simulink model "gtm_design"  (R2021b)
settings: Solver=ode15s  StartTime=0.0  StopTime=15  FixedStep=0.005  MaxStep=0.005  MinStep=0.0025
StopFcn:
  | MWSout=grabmws(bdroot);
  | MWSout.lastrun=datestr(now);
values from neighbouring files (symbols this model uses):
  s = tf('s')    [SingleDOF.m]    (also in main.m; newmain.m)
undefined symbols (not defined in the file or in its folder): Aero, aftfuel, aftfuel_pos, AILL, AILLC, AILR, AILRC, alpha_deg, altitude_ft, Ax_g, Ay_g, Az_g, b, beta_deg, bias, BRAKEC, Cbar, cg_pos0, cg_shift_gear, DamageCase, DamageModels, DamageOnsetTime, Earth, ELLIB, ELLIBC, ELLOB, ELLOBC, ELRIB, ELRIBC, ELROB, ELROBC, engl_ang, engl_pos, engr_ang, engr_pos, FLAPLIB, FLAPLIC, FLAPLOB, FLAPLOC, FLAPRIB, FLAPRIC, FLAPROB, FLAPROC, ft, FuelUsed_Init, fwdfuel, fwdfuel_pos, GEAR, GEARC, Inertia0, Inertia_shift_gear, Ixx_model, Iyy_model, Izz_model, KTAS, LandingGear, LengON, LinearizeModeOn, NAV_altitude_m, NAV_latitude_deg ... (+51)
libraries: simulink_extras x64, simulink_need_slupdate x30, LPVBlockLibrary x23, aerolibconvert2 x6, aerolibtransform2 x5, uavalgslib x4, UserContent_lib x3, simulink x3, robotcorelib x1, uavutilslib x1
(part 7 of 8)

== system gtm_design/GTM_T2/Sensors/Surface Pots/Sensor Model5 ==
  In1 : Inport
  Add : Sum  Inputs=+++
  Gain : Gain  Gain=scf
  Gear1 : Constant  Value=bias
  Gear2 : Constant  Value=noise_on
  Noise_on : Switch  Threshold=0.5  SaturateOnIntegerOverflow=on  InputSameDT=on
  White Noise : RandomNumber  Variance=sigma*sigma  Seed=round(seed*rand(1))  SampleTime=Timestep
  Out1 : Outport
  wires:
  Noise_on/1 -> Out1/1
  Gear2/1 -> Noise_on/2
  White Noise/1 -> Add/1
  Add/1 -> Noise_on/1
  Gear1/1 -> Add/2
  Gain/1 -> Add/3
  In1/1 -> Noise_on/3, Gain/1

== system gtm_design/GTM_T2/Sensors/Surface Pots/Surface Labels ==
  I : Inport
  Bus Creator : BusCreator  Inputs=12
  Demux : Demux  Outputs=12
  O : Outport
  wires:
  Bus Creator/1 -> O/1
  Demux/12 -> Bus Creator/12  "FLAPROB"
  Demux/11 -> Bus Creator/11  "FLAPRIB"
  Demux/10 -> Bus Creator/10  "FLAPLOB"
  Demux/9 -> Bus Creator/9  "FLAPLIB"
  Demux/8 -> Bus Creator/8  "RUDL"
  Demux/7 -> Bus Creator/7  "RUDU"
  Demux/6 -> Bus Creator/6  "AILR"
  Demux/5 -> Bus Creator/5  "AILL"
  Demux/4 -> Bus Creator/4  "ELRIB"
  Demux/3 -> Bus Creator/3  "ELROB"
  Demux/2 -> Bus Creator/2  "ELLIB"
  Demux/1 -> Bus Creator/1  "ELLOB"
  I/1 -> Demux/1

== system gtm_design/GTM_T2/TransportDelay/AntiAliasing/First Order Filter Continuous ==
  In : Inport
  Constant : Constant  Value=tau
  Divide : Product  Inputs=*/
  Integrator : Integrator  InitialConditionSource=external
  Sum : Sum  Inputs=-+|  InputSameDT=on  SaturateOnIntegerOverflow=on  OutDataTypeStr=Inherit: Same as first input
  Out : Outport
  wires:
  Constant/1 -> Divide/2
  Sum/1 -> Divide/1  "Error"
  In/1 -> Integrator/2, Sum/2
  Integrator/1 -> Out/1, Sum/1  "Y"
  Divide/1 -> Integrator/1  "Ydot"

== system gtm_design/GTM_T2/TransportDelay/Transport Delay on Bus/BusDelay ==
  In1 : Inport
  Bus Assignment : BusAssignment  AssignedSignals=alpha_deg,beta_deg,qbar_psf,KTAS,TEMPAMB_degF,altitude_ft
  Bus Selector1 : BusSelector  OutputSignals=alpha_deg,beta_deg,qbar_psf,KTAS,TEMPAMB_degF,altitude_ft  OutputAsBus=on
  Bus to Vector : BusToVector
  Demux : Demux  Outputs=6
  TimeDelay with IC feedthrough : Subsystem  mask{TimeDelay=15e-3}
      mask prompts: TimeDelay "Time Delay (sec)"
      mask help:
      | Implements Continuous Time Transport Delay with initial
      | outputs set to feedthrough with no delay.
      |
      |   output = input;   for t<TimeDelay
      |   output = input(t-tdelay); for t>=TimeDelay
  Out1 : Outport
  wires:
  In1/1 -> Bus Assignment/1, Bus Selector1/1
  Bus Selector1/1 -> Bus to Vector/1
  Bus to Vector/1 -> TimeDelay with IC feedthrough/1(I)
  TimeDelay with IC feedthrough/1(O) -> Demux/1
  Demux/1 -> Bus Assignment/2
  Demux/2 -> Bus Assignment/3
  Demux/3 -> Bus Assignment/4
  Demux/4 -> Bus Assignment/5
  Demux/5 -> Bus Assignment/6
  Demux/6 -> Bus Assignment/7
  Bus Assignment/1 -> Out1/1

== system gtm_design/GTM_T2/TransportDelay/Transport Delay on Bus/BusDelay1 ==
  In1 : Inport
  Bus Assignment : BusAssignment  AssignedSignals=phi_deg,theta_deg,psi_deg,NAV_latitude_deg,NAV_longitude_deg,NAV_altitude_m,NAV_Vn_mps,NAV_Ve_mps,NAV_Vu_mps
  Bus Selector1 : BusSelector  OutputSignals=phi_deg,theta_deg,psi_deg,NAV_latitude_deg,NAV_longitude_deg,NAV_altitude_m,NAV_Vn_mps,NAV_Ve_mps,NAV_Vu_mps  OutputAsBus=on
  Bus to Vector : BusToVector
  Demux : Demux  Outputs=9
  TimeDelay with IC feedthrough : Subsystem  mask{TimeDelay=15e-3}
      mask prompts: TimeDelay "Time Delay (sec)"
      mask help:
      | Implements Continuous Time Transport Delay with initial
      | outputs set to feedthrough with no delay.
      |
      |   output = input;   for t<TimeDelay
      |   output = input(t-tdelay); for t>=TimeDelay
  Out1 : Outport
  wires:
  In1/1 -> Bus Assignment/1, Bus Selector1/1
  Bus Selector1/1 -> Bus to Vector/1
  Bus to Vector/1 -> TimeDelay with IC feedthrough/1(I)
  TimeDelay with IC feedthrough/1(O) -> Demux/1
  Demux/1 -> Bus Assignment/2
  Demux/2 -> Bus Assignment/3
  Demux/3 -> Bus Assignment/4
  Demux/4 -> Bus Assignment/5
  Demux/5 -> Bus Assignment/6
  Demux/6 -> Bus Assignment/7
  Bus Assignment/1 -> Out1/1
  Demux/7 -> Bus Assignment/8
  Demux/8 -> Bus Assignment/9
  Demux/9 -> Bus Assignment/10

== system gtm_design/GTM_T2/TransportDelay/Transport Delay on Bus/BusDelay2 ==
  In1 : Inport
  Bus Assignment : BusAssignment  AssignedSignals=p_deg,q_deg,r_deg,Ax_g,Ay_g,Az_g
  Bus Selector1 : BusSelector  OutputSignals=p_deg,q_deg,r_deg,Ax_g,Ay_g,Az_g  OutputAsBus=on
  Bus to Vector : BusToVector
  Demux : Demux  Outputs=6
  TimeDelay with IC feedthrough : Subsystem  mask{TimeDelay=15e-3}
      mask prompts: TimeDelay "Time Delay (sec)"
      mask help:
      | Implements Continuous Time Transport Delay with initial
      | outputs set to feedthrough with no delay.
      |
      |   output = input;   for t<TimeDelay
      |   output = input(t-tdelay); for t>=TimeDelay
  Out1 : Outport
  wires:
  In1/1 -> Bus Assignment/1, Bus Selector1/1
  Bus Selector1/1 -> Bus to Vector/1
  Bus to Vector/1 -> TimeDelay with IC feedthrough/1(I)
  TimeDelay with IC feedthrough/1(O) -> Demux/1
  Demux/1 -> Bus Assignment/2
  Demux/2 -> Bus Assignment/3
  Demux/3 -> Bus Assignment/4
  Demux/4 -> Bus Assignment/5
  Demux/5 -> Bus Assignment/6
  Demux/6 -> Bus Assignment/7
  Bus Assignment/1 -> Out1/1

== system gtm_design/GTM_T2/TransportDelay/Transport Delay on Bus/BusDelay3 ==
  In1 : Inport
  Bus Assignment : BusAssignment  AssignedSignals=ELLOB,ELLIB,ELROB,ELRIB,AILL,AILR,RUDU,RUDL,FLAPLIB,FLAPLOB,FLAPRIB,FLAPROB
  Bus Selector1 : BusSelector  OutputSignals=ELLOB,ELLIB,ELROB,ELRIB,AILL,AILR,RUDU,RUDL,FLAPLIB,FLAPLOB,FLAPRIB,FLAPROB  OutputAsBus=on
  Bus to Vector : BusToVector
  Demux : Demux  Outputs=12
  TimeDelay with IC feedthrough : Subsystem  mask{TimeDelay=15e-3}
      mask prompts: TimeDelay "Time Delay (sec)"
      mask help:
      | Implements Continuous Time Transport Delay with initial
      | outputs set to feedthrough with no delay.
      |
      |   output = input;   for t<TimeDelay
      |   output = input(t-tdelay); for t>=TimeDelay
  Out1 : Outport
  wires:
  In1/1 -> Bus Assignment/1, Bus Selector1/1
  Bus Selector1/1 -> Bus to Vector/1
  Bus to Vector/1 -> TimeDelay with IC feedthrough/1(I)
  TimeDelay with IC feedthrough/1(O) -> Demux/1
  Bus Assignment/1 -> Out1/1
  Demux/1 -> Bus Assignment/2
  Demux/2 -> Bus Assignment/3
  Demux/3 -> Bus Assignment/4
  Demux/4 -> Bus Assignment/5
  Demux/5 -> Bus Assignment/6
  Demux/6 -> Bus Assignment/7
  Demux/7 -> Bus Assignment/8
  Demux/8 -> Bus Assignment/9
  Demux/9 -> Bus Assignment/10
  Demux/10 -> Bus Assignment/11
  Demux/11 -> Bus Assignment/12
  Demux/12 -> Bus Assignment/13

== system gtm_design/GTM_T2/TransportDelay/Transport Delay on Bus/BusDelay4 ==
  In1 : Inport
  Bus Assignment : BusAssignment  AssignedSignals=RPML,PUMPVL,RPMR,PUMPVR
  Bus Selector1 : BusSelector  OutputSignals=RPML,PUMPVL,RPMR,PUMPVR  OutputAsBus=on
  Bus to Vector : BusToVector
  Demux : Demux
  TimeDelay with IC feedthrough : Subsystem  mask{TimeDelay=15e-3}
      mask prompts: TimeDelay "Time Delay (sec)"
      mask help:
      | Implements Continuous Time Transport Delay with initial
      | outputs set to feedthrough with no delay.
      |
      |   output = input;   for t<TimeDelay
      |   output = input(t-tdelay); for t>=TimeDelay
  Out1 : Outport
  wires:
  In1/1 -> Bus Assignment/1, Bus Selector1/1
  Bus Selector1/1 -> Bus to Vector/1
  Bus to Vector/1 -> TimeDelay with IC feedthrough/1(I)
  TimeDelay with IC feedthrough/1(O) -> Demux/1
  Demux/1 -> Bus Assignment/2
  Demux/2 -> Bus Assignment/3
  Demux/3 -> Bus Assignment/4
  Demux/4 -> Bus Assignment/5
  Bus Assignment/1 -> Out1/1

== system gtm_design/GTM_T2/TransportDelay/Transport Delay on Bus1/BusDelay ==
  In1 : Inport
  Bus Assignment : BusAssignment  AssignedSignals=THROTLC,THROTRC,ELLOBC,ELLIBC,ELROBC,ELRIBC,AILLC,AILRC,RUDUPC,RUDLOC,SPLLIBC,SPLLOBC,SPLRIBC,SPLROBC,FLAPLIC,FLAPLOC,FLAPRIC,FLAPROC,GEARC,BRAKEC,STEERC
  Bus Selector1 : BusSelector  OutputSignals=THROTLC,THROTRC,ELLOBC,ELLIBC,ELROBC,ELRIBC,AILLC,AILRC,RUDUPC,RUDLOC,SPLLIBC,SPLLOBC,SPLRIBC,SPLROBC,FLAPLIC,FLAPLOC,FLAPRIC,FLAPROC,GEARC,BRAKEC,STEERC  OutputAsBus=on
  Bus to Vector : BusToVector
  Demux : Demux  Outputs=21
  Transport Delay : TransportDelay  DelayTime=5e-3
      settings: AttributesFormatString=%<DelayTime>
  Out1 : Outport
  wires:
  In1/1 -> Bus Assignment/1, Bus Selector1/1
  Bus Selector1/1 -> Bus to Vector/1
  Bus to Vector/1 -> Transport Delay/1
  Transport Delay/1 -> Demux/1
  Demux/1 -> Bus Assignment/2
  Demux/2 -> Bus Assignment/3
  Demux/3 -> Bus Assignment/4
  Demux/4 -> Bus Assignment/5
  Demux/5 -> Bus Assignment/6
  Demux/6 -> Bus Assignment/7
  Bus Assignment/1 -> Out1/1
  Demux/7 -> Bus Assignment/8
  Demux/8 -> Bus Assignment/9
  Demux/9 -> Bus Assignment/10
  Demux/10 -> Bus Assignment/11
  Demux/11 -> Bus Assignment/12
  Demux/12 -> Bus Assignment/13
  Demux/13 -> Bus Assignment/14
  Demux/14 -> Bus Assignment/15
  Demux/15 -> Bus Assignment/16
  Demux/16 -> Bus Assignment/17
  Demux/17 -> Bus Assignment/18
  Demux/18 -> Bus Assignment/19
  Demux/19 -> Bus Assignment/20
  Demux/20 -> Bus Assignment/21
  Demux/21 -> Bus Assignment/22

== system gtm_design/GTM_T2/A//C parameters/Inertia//Mass//CG Shift/FuelBurnEffects/Polyval ==
  In1 : Inport
  Embedded MATLAB Function : MATLAB Function  TreatAsAtomicUnit=on
  Out1 : Outport
  wires:
  In1/1 -> Embedded MATLAB Function/1(u)
  Embedded MATLAB Function/1(y) -> Out1/1

== system gtm_design/GTM_T2/A//C parameters/Inertia//Mass//CG Shift/FuelBurnEffects/Polyval1 ==
  In1 : Inport
  Embedded MATLAB Function : MATLAB Function  TreatAsAtomicUnit=on
  Out1 : Outport
  wires:
  In1/1 -> Embedded MATLAB Function/1(u)
  Embedded MATLAB Function/1(y) -> Out1/1

== system gtm_design/GTM_T2/A//C parameters/Inertia//Mass//CG Shift/FuelBurnEffects/Polyval2 ==
  In1 : Inport
  Embedded MATLAB Function : MATLAB Function  TreatAsAtomicUnit=on
  Out1 : Outport
  wires:
  In1/1 -> Embedded MATLAB Function/1(u)
  Embedded MATLAB Function/1(y) -> Out1/1

== system gtm_design/GTM_T2/Actuators/InputModification for Trimming/LinearizeMode:DetlasOnTrimBias/Surface Allocation For Linearizing ==
  I : Inport
  BiasSurfs : Subsystem
  Demux : Demux  Outputs=19
  Gain1 : Gain  Gain=-1
  Ground1 : Ground
  Ground2 : Ground
  Ground5 : Ground
  Mux : Mux  Inputs=22
  O : Outport
  wires:
  BiasSurfs/1(cmds) -> O/1
  I/1 -> Demux/1
  Mux/1 -> BiasSurfs/1(dCmd)
  Ground1/1 -> Mux/18  "dgear"
  Ground2/1 -> Mux/19  "dbrake"
  Ground5/1 -> Mux/22  "dSteer"
  Demux/1 -> Mux/1  "dElevatorLOB"
  Demux/2 -> Mux/2  "dElevatorLIB"
  Demux/3 -> Mux/3  "dElevatorROB"
  Demux/4 -> Mux/4  "dElevatorRIB"
  Demux/5 -> Gain1/1  "dAileronL"
  Demux/6 -> Mux/6  "dAileronR"
  Demux/7 -> Mux/7  "dRudderUpper"
  Demux/8 -> Mux/8  "dRudderLower"
  Demux/9 -> Mux/9  "dSpoilerLOB"
  Demux/10 -> Mux/10  "dSpoilerLIB"
  Demux/11 -> Mux/11  "dSpoilerRIB"
  Demux/12 -> Mux/12  "dSpoilerROB"
  Demux/13 -> Mux/13  "dFlapLIB"
  Demux/14 -> Mux/14  "dFlapLOB"
  Demux/15 -> Mux/15  "dFlapRIB"
  Demux/16 -> Mux/16  "dFlapROB"
  Demux/17 -> Mux/17  "dStabilizer"
  Demux/18 -> Mux/20  "dThrottleL"
  Demux/19 -> Mux/21  "dThrottleR"
  Gain1/1 -> Mux/5  "dAileronL"

== system gtm_design/GTM_T2/Actuators/InputModification for Trimming/TrimMode: DriveFromTopLevel/Force Consistent Sample Time on Bus ==
  In1 : Inport
  Bus to Vector : BusToVector
  Map4 : Gain
  Out1 : Outport
  wires:
  In1/1 -> Bus to Vector/1
  Map4/1 -> Out1/1
  Bus to Vector/1 -> Map4/1

== system gtm_design/GTM_T2/Actuators/InputModification for Trimming/TrimMode: DriveFromTopLevel/InitializeBus ==
  Bus Creator : BusCreator  Inputs=22
  Constant : Constant  Value=zeros(22,1)
  Demux : Demux  Outputs=22
  O : Outport
  wires:
  Constant/1 -> Demux/1
  Demux/18 -> Bus Creator/18  "GEAR"
  Demux/19 -> Bus Creator/19  "BRAKE"
  Demux/20 -> Bus Creator/20  "THROTL"
  Demux/21 -> Bus Creator/21  "THROTR"
  Demux/22 -> Bus Creator/22  "STEER"
  Demux/17 -> Bus Creator/17  "STAB"
  Bus Creator/1 -> O/1
  Demux/2 -> Bus Creator/2  "ELLIB"
  Demux/3 -> Bus Creator/3  "ELROB"
  Demux/4 -> Bus Creator/4  "ELRIB"
  Demux/5 -> Bus Creator/5  "AILL"
  Demux/6 -> Bus Creator/6  "AILR"
  Demux/7 -> Bus Creator/7  "RUDU"
  Demux/8 -> Bus Creator/8  "RUDL"
  Demux/9 -> Bus Creator/9  "SPLLIB"
  Demux/10 -> Bus Creator/10  "SPLLOB"
  Demux/11 -> Bus Creator/11  "SPLRIB"
  Demux/12 -> Bus Creator/12  "SPLROB"
  Demux/13 -> Bus Creator/13  "FLAPLIB"
  Demux/14 -> Bus Creator/14  "FLAPLOB"
  Demux/15 -> Bus Creator/15  "FLAPRIB"
  Demux/16 -> Bus Creator/16  "FLAPROB"
  Demux/1 -> Bus Creator/1  "ELLOB"

== system gtm_design/GTM_T2/Actuators/InputModification for Trimming/TrimMode: DriveFromTopLevel/MapPitchSurf ==
  UseStab : Inport
  In : Inport  Port=2
  Merge : Merge
  Switch Case : SwitchCase
  UseElevatorToTrim : Subsystem  TreatAsAtomicUnit=on
  UseStabToTrim : Subsystem  TreatAsAtomicUnit=on
  Out : Outport
  wires:
  UseElevatorToTrim/1(Out) -> Merge/1
  UseStabToTrim/1(Out1) -> Merge/2
  In/1 -> UseStabToTrim/1(In), UseElevatorToTrim/1(In)
  Merge/1 -> Out/1
  Switch Case/2 -> UseElevatorToTrim/Action
  UseStab/1 -> Switch Case/1
  Switch Case/1 -> UseStabToTrim/Action

== system gtm_design/GTM_T2/Aero/Basic Airframe/DamageEffects/Switch Case Action Subsystem ==
  alpha : Inport
  beta : Inport  Port=2
  damage_case : Inport  Port=3
  Action Port : ActionPort  ActionPortLabel=case [ 1 2 3 4 5 6 ]:
  AlphaLookup : PreLookup  BreakpointsData=Aero.dC6_damage.bas.alpha  BeginIndexSearchUsingPreviousIndexResult=on  ExtrapMethod=Linear
  BetaLookup : PreLookup  BreakpointsData=Aero.dC6_damage.bas.beta  ExtrapMethod=Linear
  Constant : Constant  Value=uint32(1)
  Constant4 : Constant  Value=[0:5]  OutDataTypeStr=uint32
  Interpolation Using Prelookup : Interpolation_n-D  NumberOfTableDimensions=4  Table=Aero.dC6_damage.bas.data  ExtrapMethod=Clip  NumSelectionDims=2
      settings: InputPortMap=u0,u1,u2,u3,u4,u5
  Subtract : Sum  Inputs=+-
  dC6_dam : Outport  InitialOutput=zeros(6,1)
  wires:
  Constant/1 -> Subtract/2
  Subtract/1 -> Interpolation Using Prelookup/5
  damage_case/1 -> Subtract/1
  BetaLookup/2 -> Interpolation Using Prelookup/4
  BetaLookup/1 -> Interpolation Using Prelookup/3
  AlphaLookup/2 -> Interpolation Using Prelookup/2
  AlphaLookup/1 -> Interpolation Using Prelookup/1
  Interpolation Using Prelookup/1 -> dC6_dam/1
  beta/1 -> BetaLookup/1
  alpha/1 -> AlphaLookup/1
  Constant4/1 -> Interpolation Using Prelookup/6

== system gtm_design/GTM_T2/Aero/Basic Airframe/DamageEffects/Switch Case Action Subsystem2 ==
  Action Port : ActionPort  ActionPortLabel=default:
  Constant4 : Constant  Value=zeros(6,1)  OutDataTypeStr=double
  Zeros : Outport  InitialOutput=zeros(6,1)
  wires:
  Constant4/1 -> Zeros/1

== system gtm_design/GTM_T2/Aero/Control Surfaces/Elevator//Stab1/RollYaw Coupling LIB ==
  I : Inport
  Gain : Gain  Gain=Kc  Multiplication=Matrix(K*u)
  O : Outport
  wires:
  Gain/1 -> O/1
  I/1 -> Gain/1

== system gtm_design/GTM_T2/Aero/Control Surfaces/Elevator//Stab1/RollYaw Coupling LOB ==
  I : Inport
  Gain : Gain  Gain=Kc  Multiplication=Matrix(K*u)
  O : Outport
  wires:
  Gain/1 -> O/1
  I/1 -> Gain/1

== system gtm_design/GTM_T2/Aero/Control Surfaces/Elevator//Stab1/RollYaw Coupling RIB ==
  I : Inport
  Gain : Gain  Gain=Kc  Multiplication=Matrix(K*u)
  O : Outport
  wires:
  Gain/1 -> O/1
  I/1 -> Gain/1

== system gtm_design/GTM_T2/Aero/Control Surfaces/Elevator//Stab1/RollYaw Coupling ROB ==
  I : Inport
  Gain : Gain  Gain=Kc  Multiplication=Matrix(K*u)
  O : Outport
  wires:
  Gain/1 -> O/1
  I/1 -> Gain/1

== system gtm_design/GTM_T2/Aero/Control Surfaces/Elevator//Stab1/Stab//Elev Table ==
  alpha_k : Inport
  alpha_f : Inport  Port=2
  beta_k : Inport  Port=3
  beta_f : Inport  Port=4
  stab_k : Inport  Port=5
  stab_f : Inport  Port=6
  elev : Inport  Port=7
  Assignment to Longitudinal : Assignment  IndexMode=Zero-based  IndexOptions=Index vector (dialog)  Indices=[0 2 4]  OutputSizes=[1 1]
  Constant : Constant  Value=zeros(6,1)
  Constant2 : Constant  Value=[0:2]  OutDataTypeStr=uint32
  Interpolation Using Prelookup : Interpolation_n-D  NumberOfTableDimensions=5  Table=Aero.dC3_ele.data  NumSelectionDims=1
      settings: InputPortMap=u0,u1,u2,u3,u4,u5,u6,u7,u8
  Prelookup4 : PreLookup  BreakpointsData=Aero.dC3_ele.elev  IndexSearchMethod=Linear search  BeginIndexSearchUsingPreviousIndexResult=on  ExtrapMethod=Linear
  dC6 : Outport
  wires:
  Constant2/1 -> Interpolation Using Prelookup/9
  Prelookup4/2 -> Interpolation Using Prelookup/8
  Prelookup4/1 -> Interpolation Using Prelookup/7
  stab_f/1 -> Interpolation Using Prelookup/6
  beta_f/1 -> Interpolation Using Prelookup/4
  alpha_f/1 -> Interpolation Using Prelookup/2
  alpha_k/1 -> Interpolation Using Prelookup/1
  beta_k/1 -> Interpolation Using Prelookup/3
  stab_k/1 -> Interpolation Using Prelookup/5
  elev/1 -> Prelookup4/1
  Constant/1 -> Assignment to Longitudinal/1
  Interpolation Using Prelookup/1 -> Assignment to Longitudinal/2
  Assignment to Longitudinal/1 -> dC6/1

== system gtm_design/GTM_T2/Aero/Control Surfaces/Elevator//Stab1/Stab//Elev Table0 ==
  alpha_k : Inport
  alpha_f : Inport  Port=2
  beta_k : Inport  Port=3
  beta_f : Inport  Port=4
  stab_k : Inport  Port=5
  stab_f : Inport  Port=6
  elev : Inport  Port=7
  Assignment to Longitudinal : Assignment  IndexMode=Zero-based  IndexOptions=Index vector (dialog)  Indices=[0 2 4]  OutputSizes=[1 1]
  Constant : Constant  Value=zeros(6,1)
  Constant2 : Constant  Value=[0:2]  OutDataTypeStr=uint32
  Interpolation Using Prelookup : Interpolation_n-D  NumberOfTableDimensions=5  Table=Aero.dC3_ele.data  NumSelectionDims=1
      settings: InputPortMap=u0,u1,u2,u3,u4,u5,u6,u7,u8
  Prelookup4 : PreLookup  BreakpointsData=Aero.dC3_ele.elev  IndexSearchMethod=Linear search  BeginIndexSearchUsingPreviousIndexResult=on  ExtrapMethod=Linear
  dC6 : Outport
  wires:
  Constant2/1 -> Interpolation Using Prelookup/9
  Prelookup4/2 -> Interpolation Using Prelookup/8
  Prelookup4/1 -> Interpolation Using Prelookup/7
  stab_f/1 -> Interpolation Using Prelookup/6
  beta_f/1 -> Interpolation Using Prelookup/4
  alpha_f/1 -> Interpolation Using Prelookup/2
  alpha_k/1 -> Interpolation Using Prelookup/1
  beta_k/1 -> Interpolation Using Prelookup/3
  stab_k/1 -> Interpolation Using Prelookup/5
  elev/1 -> Prelookup4/1
  Constant/1 -> Assignment to Longitudinal/1
  Interpolation Using Prelookup/1 -> Assignment to Longitudinal/2
  Assignment to Longitudinal/1 -> dC6/1

== system gtm_design/GTM_T2/Aero/Control Surfaces/Elevator//Stab1/Stab//Elev Table1 ==
  alpha_k : Inport
  alpha_f : Inport  Port=2
  beta_k : Inport  Port=3
  beta_f : Inport  Port=4
  stab_k : Inport  Port=5
  stab_f : Inport  Port=6
  elev : Inport  Port=7
  Assignment to Longitudinal : Assignment  IndexMode=Zero-based  IndexOptions=Index vector (dialog)  Indices=[0 2 4]  OutputSizes=[1 1]
  Constant : Constant  Value=zeros(6,1)
  Constant2 : Constant  Value=[0:2]  OutDataTypeStr=uint32
  Interpolation Using Prelookup : Interpolation_n-D  NumberOfTableDimensions=5  Table=Aero.dC3_ele.data  NumSelectionDims=1
      settings: InputPortMap=u0,u1,u2,u3,u4,u5,u6,u7,u8
  Prelookup4 : PreLookup  BreakpointsData=Aero.dC3_ele.elev  IndexSearchMethod=Linear search  BeginIndexSearchUsingPreviousIndexResult=on  ExtrapMethod=Linear
  dC6 : Outport
  wires:
  Constant2/1 -> Interpolation Using Prelookup/9
  Prelookup4/2 -> Interpolation Using Prelookup/8
  Prelookup4/1 -> Interpolation Using Prelookup/7
  stab_f/1 -> Interpolation Using Prelookup/6
  beta_f/1 -> Interpolation Using Prelookup/4
  alpha_f/1 -> Interpolation Using Prelookup/2
  alpha_k/1 -> Interpolation Using Prelookup/1
  beta_k/1 -> Interpolation Using Prelookup/3
  stab_k/1 -> Interpolation Using Prelookup/5
  elev/1 -> Prelookup4/1
  Constant/1 -> Assignment to Longitudinal/1
  Interpolation Using Prelookup/1 -> Assignment to Longitudinal/2
  Assignment to Longitudinal/1 -> dC6/1

== system gtm_design/GTM_T2/Aero/Control Surfaces/Elevator//Stab1/Stab//Elev Table2 ==
  alpha_k : Inport
  alpha_f : Inport  Port=2
  beta_k : Inport  Port=3
  beta_f : Inport  Port=4
  stab_k : Inport  Port=5
  stab_f : Inport  Port=6
  elev : Inport  Port=7
  Assignment to Longitudinal : Assignment  IndexMode=Zero-based  IndexOptions=Index vector (dialog)  Indices=[0 2 4]  OutputSizes=[1 1]
  Constant : Constant  Value=zeros(6,1)
  Constant2 : Constant  Value=[0:2]  OutDataTypeStr=uint32
  Interpolation Using Prelookup : Interpolation_n-D  NumberOfTableDimensions=5  Table=Aero.dC3_ele.data  NumSelectionDims=1
      settings: InputPortMap=u0,u1,u2,u3,u4,u5,u6,u7,u8
  Prelookup4 : PreLookup  BreakpointsData=Aero.dC3_ele.elev  IndexSearchMethod=Linear search  BeginIndexSearchUsingPreviousIndexResult=on  ExtrapMethod=Linear
  dC6 : Outport
  wires:
  Constant2/1 -> Interpolation Using Prelookup/9
  Prelookup4/2 -> Interpolation Using Prelookup/8
  Prelookup4/1 -> Interpolation Using Prelookup/7
  stab_f/1 -> Interpolation Using Prelookup/6
  beta_f/1 -> Interpolation Using Prelookup/4
  alpha_f/1 -> Interpolation Using Prelookup/2
  alpha_k/1 -> Interpolation Using Prelookup/1
  beta_k/1 -> Interpolation Using Prelookup/3
  stab_k/1 -> Interpolation Using Prelookup/5
  elev/1 -> Prelookup4/1
  Constant/1 -> Assignment to Longitudinal/1
  Interpolation Using Prelookup/1 -> Assignment to Longitudinal/2
  Assignment to Longitudinal/1 -> dC6/1

== system gtm_design/GTM_T2/Aero/Control Surfaces/Elevator//Stab1/Stab//Elev Table3 ==
  alpha_k : Inport
  alpha_f : Inport  Port=2
  beta_k : Inport  Port=3
  beta_f : Inport  Port=4
  stab_k : Inport  Port=5
  stab_f : Inport  Port=6
  elev : Inport  Port=7
  Assignment to Longitudinal : Assignment  IndexMode=Zero-based  IndexOptions=Index vector (dialog)  Indices=[0 2 4]  OutputSizes=[1 1]
  Constant : Constant  Value=zeros(6,1)
  Constant2 : Constant  Value=[0:2]  OutDataTypeStr=uint32
  Interpolation Using Prelookup : Interpolation_n-D  NumberOfTableDimensions=5  Table=Aero.dC3_ele.data  NumSelectionDims=1
      settings: InputPortMap=u0,u1,u2,u3,u4,u5,u6,u7,u8
  Prelookup4 : PreLookup  BreakpointsData=Aero.dC3_ele.elev  IndexSearchMethod=Linear search  BeginIndexSearchUsingPreviousIndexResult=on  ExtrapMethod=Linear
  dC6 : Outport
  wires:
  Constant2/1 -> Interpolation Using Prelookup/9
  Prelookup4/2 -> Interpolation Using Prelookup/8
  Prelookup4/1 -> Interpolation Using Prelookup/7
  stab_f/1 -> Interpolation Using Prelookup/6
  beta_f/1 -> Interpolation Using Prelookup/4
  alpha_f/1 -> Interpolation Using Prelookup/2
  alpha_k/1 -> Interpolation Using Prelookup/1
  beta_k/1 -> Interpolation Using Prelookup/3
  stab_k/1 -> Interpolation Using Prelookup/5
  elev/1 -> Prelookup4/1
  Constant/1 -> Assignment to Longitudinal/1
  Interpolation Using Prelookup/1 -> Assignment to Longitudinal/2
  Assignment to Longitudinal/1 -> dC6/1

== system gtm_design/GTM_T2/Aero/Control Surfaces/Rudder/Gains ==
  dC6_in : Inport
  Product : Product  RndMeth=Zero
  gains : Constant  Value=gains
  dC6 : Outport
  wires:
  dC6_in/1 -> Product/1
  Product/1 -> dC6/1
  gains/1 -> Product/2

== system gtm_design/GTM_T2/Aero/Control Surfaces/Rudder/Gains1 ==
  dC6_in : Inport
  Product : Product  RndMeth=Zero
  gains : Constant  Value=gains
  dC6 : Outport
  wires:
  gains/1 -> Product/2
  Product/1 -> dC6/1
  dC6_in/1 -> Product/1

== system gtm_design/GTM_T2/Aero/Control Surfaces/Rudder/Lower Rudder ==
  alpha : Inport
  beta : Inport  Port=2
  rud : Inport  Port=3
  Abs : Abs
  Assignment to lateral : Assignment  IndexMode=Zero-based  IndexOptions=Index vector (dialog)  Indices=[1 3 5]  OutputSizes=[1 1]
  Constant : Constant  Value=-1
  Constant1 : Constant
  Constant2 : Constant  Value=[0:5]  OutDataTypeStr=uint32
  Constant3 : Constant  Value=ones(6,1)
  Gain : Gain  Gain=-1
  Interpolation Using Prelookup : Interpolation_n-D  NumberOfTableDimensions=4  Table=Aero.dC6_rud.data  NumSelectionDims=1
      settings: InputPortMap=u0,u1,u2,u3,u4,u5,u6
  Prelookup : PreLookup  BreakpointsData=Aero.dC6_rud.alpha  IndexSearchMethod=Linear search  BeginIndexSearchUsingPreviousIndexResult=on  ExtrapMethod=Linear
  Prelookup1 : PreLookup  BreakpointsData=Aero.dC6_rud.beta  IndexSearchMethod=Linear search  BeginIndexSearchUsingPreviousIndexResult=on  ExtrapMethod=Linear
  Prelookup2 : PreLookup  BreakpointsData=Aero.dC6_rud.rud  IndexSearchMethod=Linear search  BeginIndexSearchUsingPreviousIndexResult=on  ExtrapMethod=Linear
  Product1 : Product  RndMeth=Zero
  Product2 : Product  RndMeth=Zero
  Switch : Switch
  dC6 : Outport
  wires:
  Interpolation Using Prelookup/1 -> Product2/1
  Assignment to lateral/1 -> Product2/2
  Constant3/1 -> Assignment to lateral/1
  Switch/1 -> Assignment to lateral/2, Product1/2
  Constant1/1 -> Switch/3
  Constant/1 -> Switch/1
  Product2/1 -> dC6/1
  beta/1 -> Product1/1
  alpha/1 -> Prelookup/1
  Gain/1 -> Prelookup2/1
  Abs/1 -> Gain/1
  rud/1 -> Switch/2, Abs/1
  Product1/1 -> Prelookup1/1
  Prelookup/1 -> Interpolation Using Prelookup/1
  Prelookup/2 -> Interpolation Using Prelookup/2
  Prelookup1/1 -> Interpolation Using Prelookup/3
  Prelookup1/2 -> Interpolation Using Prelookup/4
  Prelookup2/1 -> Interpolation Using Prelookup/5
  Prelookup2/2 -> Interpolation Using Prelookup/6
  Constant2/1 -> Interpolation Using Prelookup/7

== system gtm_design/GTM_T2/Aero/Control Surfaces/Rudder/Upper Rudder ==
  alpha : Inport
  beta : Inport  Port=2
  rud : Inport  Port=3
  Abs : Abs
  Assignment to lateral : Assignment  IndexMode=Zero-based  IndexOptions=Index vector (dialog)  Indices=[1 3 5]  OutputSizes=[1 1]
  Constant : Constant  Value=-1
  Constant1 : Constant
  Constant2 : Constant  Value=[0:5]  OutDataTypeStr=uint32
  Constant3 : Constant  Value=ones(6,1)
  Gain : Gain  Gain=-1
  Interpolation Using Prelookup : Interpolation_n-D  NumberOfTableDimensions=4  Table=Aero.dC6_rud.data  NumSelectionDims=1
      settings: InputPortMap=u0,u1,u2,u3,u4,u5,u6
  Prelookup : PreLookup  BreakpointsData=Aero.dC6_rud.alpha  IndexSearchMethod=Linear search  BeginIndexSearchUsingPreviousIndexResult=on  ExtrapMethod=Linear
  Prelookup1 : PreLookup  BreakpointsData=Aero.dC6_rud.beta  IndexSearchMethod=Linear search  BeginIndexSearchUsingPreviousIndexResult=on  ExtrapMethod=Linear
  Prelookup2 : PreLookup  BreakpointsData=Aero.dC6_rud.rud  IndexSearchMethod=Linear search  BeginIndexSearchUsingPreviousIndexResult=on  ExtrapMethod=Linear
  Product1 : Product  RndMeth=Zero
  Product2 : Product  RndMeth=Zero
  Switch : Switch
  dC6 : Outport
  wires:
  Constant2/1 -> Interpolation Using Prelookup/7
  Prelookup2/2 -> Interpolation Using Prelookup/6
  Prelookup2/1 -> Interpolation Using Prelookup/5
  Prelookup1/2 -> Interpolation Using Prelookup/4
  Prelookup1/1 -> Interpolation Using Prelookup/3
  Prelookup/2 -> Interpolation Using Prelookup/2
  Prelookup/1 -> Interpolation Using Prelookup/1
  Product1/1 -> Prelookup1/1
  rud/1 -> Abs/1, Switch/2
  Abs/1 -> Gain/1
  Gain/1 -> Prelookup2/1
  alpha/1 -> Prelookup/1
  beta/1 -> Product1/1
  Product2/1 -> dC6/1
  Constant/1 -> Switch/1
  Constant1/1 -> Switch/3
  Switch/1 -> Product1/2, Assignment to lateral/2
  Constant3/1 -> Assignment to lateral/1
  Assignment to lateral/1 -> Product2/2
  Interpolation Using Prelookup/1 -> Product2/1

== system gtm_design/GTM_T2/Aero/Control Surfaces/Spoilers/Gains1 ==
  dC6_in : Inport
  Product : Product  RndMeth=Zero
  gains : Constant  Value=gains
  dC6 : Outport
  wires:
  dC6_in/1 -> Product/1
  Product/1 -> dC6/1
  gains/1 -> Product/2

== system gtm_design/GTM_T2/Aero/Control Surfaces/Spoilers/Gains2 ==
  dC6_in : Inport
  Product : Product  RndMeth=Zero
  gains : Constant  Value=gains
  dC6 : Outport
  wires:
  gains/1 -> Product/2
  Product/1 -> dC6/1
  dC6_in/1 -> Product/1

== system gtm_design/GTM_T2/Aero/Control Surfaces/Spoilers/Gains3 ==
  dC6_in : Inport
  Product : Product  RndMeth=Zero
  gains : Constant  Value=gains
  dC6 : Outport
  wires:
  gains/1 -> Product/2
  Product/1 -> dC6/1
  dC6_in/1 -> Product/1

== system gtm_design/GTM_T2/Aero/Control Surfaces/Spoilers/Gains4 ==
  dC6_in : Inport
  Product : Product  RndMeth=Zero
  gains : Constant  Value=gains
  dC6 : Outport
  wires:
  dC6_in/1 -> Product/1
  Product/1 -> dC6/1
  gains/1 -> Product/2

== system gtm_design/GTM_T2/Aero/Control Surfaces/Spoilers/InboardSpoilers ==
  alpha : Inport
  beta : Inport  Port=2
  SPLLIB : Inport  Port=3
  SPLRIB : Inport  Port=4
  Constant1 : Constant  Value=[0:5]  OutDataTypeStr=uint32
  Constant3 : Constant  Value=[0:5]  OutDataTypeStr=uint32
  Gain2 : Gain  Gain=-1
  Interpolation Using Prelookup : Interpolation_n-D  NumberOfTableDimensions=4  Table=Aero.dC6_spo.data  NumSelectionDims=1
      settings: InputPortMap=u0,u1,u2,u3,u4,u5,u6
  Interpolation Using Prelookup1 : Interpolation_n-D  NumberOfTableDimensions=4  Table=Aero.dC6_spo.data  NumSelectionDims=1
      settings: InputPortMap=u0,u1,u2,u3,u4,u5,u6
  Negate Lateral : Gain  Gain=[1 -1 1 -1 1 -1]
  Prelookup1 : PreLookup  BreakpointsData=Aero.dC6_spo.alpha  IndexSearchMethod=Linear search  BeginIndexSearchUsingPreviousIndexResult=on  ExtrapMethod=Linear
  Prelookup2 : PreLookup  BreakpointsData=Aero.dC6_spo.beta  IndexSearchMethod=Linear search  BeginIndexSearchUsingPreviousIndexResult=on  ExtrapMethod=Linear
  Prelookup3 : PreLookup  BreakpointsData=Aero.dC6_spo.spo  IndexSearchMethod=Linear search  BeginIndexSearchUsingPreviousIndexResult=on  ExtrapMethod=Linear
  Prelookup4 : PreLookup  BreakpointsData=Aero.dC6_spo.beta  IndexSearchMethod=Linear search  BeginIndexSearchUsingPreviousIndexResult=on  ExtrapMethod=Linear
  Prelookup5 : PreLookup  BreakpointsData=Aero.dC6_spo.spo  IndexSearchMethod=Linear search  BeginIndexSearchUsingPreviousIndexResult=on  ExtrapMethod=Linear
  Left : Outport
  Right : Outport  Port=2
  wires:
  Gain2/1 -> Prelookup2/1
  Negate Lateral/1 -> Left/1
  Interpolation Using Prelookup1/1 -> Right/1
  SPLRIB/1 -> Prelookup5/1
  beta/1 -> Gain2/1, Prelookup4/1
  alpha/1 -> Prelookup1/1
  SPLLIB/1 -> Prelookup3/1
  Prelookup1/1 -> Interpolation Using Prelookup/1, Interpolation Using Prelookup1/1
  Prelookup1/2 -> Interpolation Using Prelookup/2, Interpolation Using Prelookup1/2
  Prelookup2/1 -> Interpolation Using Prelookup/3
  Prelookup2/2 -> Interpolation Using Prelookup/4
  Prelookup3/1 -> Interpolation Using Prelookup/5
  Prelookup3/2 -> Interpolation Using Prelookup/6
  Constant3/1 -> Interpolation Using Prelookup/7
  Prelookup4/1 -> Interpolation Using Prelookup1/3
  Prelookup4/2 -> Interpolation Using Prelookup1/4
  Prelookup5/1 -> Interpolation Using Prelookup1/5
  Prelookup5/2 -> Interpolation Using Prelookup1/6
  Constant1/1 -> Interpolation Using Prelookup1/7
  Interpolation Using Prelookup/1 -> Negate Lateral/1

== system gtm_design/GTM_T2/Aero/Control Surfaces/Spoilers/OutboardSpoilers ==
  alpha : Inport
  beta : Inport  Port=2
  SPLLIB : Inport  Port=3
  SPLRIB : Inport  Port=4
  Constant1 : Constant  Value=[0:5]  OutDataTypeStr=uint32
  Constant3 : Constant  Value=[0:5]  OutDataTypeStr=uint32
  Gain2 : Gain  Gain=-1
  Interpolation Using Prelookup : Interpolation_n-D  NumberOfTableDimensions=4  Table=Aero.dC6_spo.data  NumSelectionDims=1
      settings: InputPortMap=u0,u1,u2,u3,u4,u5,u6
  Interpolation Using Prelookup1 : Interpolation_n-D  NumberOfTableDimensions=4  Table=Aero.dC6_spo.data  NumSelectionDims=1
      settings: InputPortMap=u0,u1,u2,u3,u4,u5,u6
  Negate Lateral : Gain  Gain=[1 -1 1 -1 1 -1]
  Prelookup1 : PreLookup  BreakpointsData=Aero.dC6_spo.alpha  IndexSearchMethod=Linear search  BeginIndexSearchUsingPreviousIndexResult=on  ExtrapMethod=Linear
  Prelookup2 : PreLookup  BreakpointsData=Aero.dC6_spo.beta  IndexSearchMethod=Linear search  BeginIndexSearchUsingPreviousIndexResult=on  ExtrapMethod=Linear
  Prelookup3 : PreLookup  BreakpointsData=Aero.dC6_spo.spo  IndexSearchMethod=Linear search  BeginIndexSearchUsingPreviousIndexResult=on  ExtrapMethod=Linear
  Prelookup4 : PreLookup  BreakpointsData=Aero.dC6_spo.beta  IndexSearchMethod=Linear search  BeginIndexSearchUsingPreviousIndexResult=on  ExtrapMethod=Linear
  Prelookup5 : PreLookup  BreakpointsData=Aero.dC6_spo.spo  IndexSearchMethod=Linear search  BeginIndexSearchUsingPreviousIndexResult=on  ExtrapMethod=Linear
  Left : Outport
  Right : Outport  Port=2
  wires:
  Interpolation Using Prelookup/1 -> Negate Lateral/1
  Constant1/1 -> Interpolation Using Prelookup1/7
  Prelookup5/2 -> Interpolation Using Prelookup1/6
  Prelookup5/1 -> Interpolation Using Prelookup1/5
  Prelookup4/2 -> Interpolation Using Prelookup1/4
  Prelookup4/1 -> Interpolation Using Prelookup1/3
  Constant3/1 -> Interpolation Using Prelookup/7
  Prelookup3/2 -> Interpolation Using Prelookup/6
  Prelookup3/1 -> Interpolation Using Prelookup/5
  Prelookup2/2 -> Interpolation Using Prelookup/4
  Prelookup2/1 -> Interpolation Using Prelookup/3
  Prelookup1/2 -> Interpolation Using Prelookup1/2, Interpolation Using Prelookup/2
  Prelookup1/1 -> Interpolation Using Prelookup1/1, Interpolation Using Prelookup/1
  SPLLIB/1 -> Prelookup3/1
  alpha/1 -> Prelookup1/1
  beta/1 -> Prelookup4/1, Gain2/1
  SPLRIB/1 -> Prelookup5/1
  Interpolation Using Prelookup1/1 -> Right/1
  Negate Lateral/1 -> Left/1
  Gain2/1 -> Prelookup2/1

== system gtm_design/GTM_T2/Aero/Dynamic Derviatives/Forced Oscillation with Damage Increments/Damage Effects-Increments ==
  alpha : Inport
  pqr : Inport  Port=2
  DamageCase : Inport  Port=3
  CY derivative increment due to rates : simulink_need_slupdate/Interpolation (n-D) using PreLookup  numDimsPopupSelect=3  explicitNumDims=2  table=squeeze(Aero.dC6_damage.ddinc.data(:,:,:,2))  interpMethod=Linear  extrapMethod=Linear  rangeErrorMode=None  NumSelectionDims=2
      settings: SourceProductBaseCode=SL
  Constant : Constant  Value=uint32(1)
  Constant1 : Constant  Value=[0:2]  OutDataTypeStr=uint32
  Data Type Conversion : DataTypeConversion  OutDataTypeStr=uint32
  PreLookup Index Search : simulink_need_slupdate/PreLookup Index Search  bpData=Aero.dC6_damage.ddinc.alpha  searchMode=Binary Search  cacheBpFlag=on  outputFlag=off  IndexDataType=uint32  extrapMode=Linear Extrapolation  rangeErrorMode=None
      settings: SourceProductBaseCode=SL
  Product : Product  RndMeth=Zero
  Subtract : Sum  Inputs=+-
  Sum of Elements : Sum  Inputs=+
  Increment : Outport
  wires:
  Subtract/1 -> CY derivative increment due to rates/2
  Data Type Conversion/1 -> Subtract/1
  Constant/1 -> Subtract/2
  Constant1/1 -> CY derivative increment due to rates/3
  PreLookup Index Search/1 -> CY derivative increment due to rates/1
  DamageCase/1 -> Data Type Conversion/1
  alpha/1 -> PreLookup Index Search/1
  CY derivative increment due to rates/1 -> Product/1
  pqr/1 -> Product/2
  Product/1 -> Sum of Elements/1
  Sum of Elements/1 -> Increment/1

== system gtm_design/GTM_T2/Aero/Dynamic Derviatives/Forced Oscillation with Damage Increments/Damage Effects-Scaling ==
  alpha : Inport
  DamageCase : Inport  Port=2
  Constant : Constant  Value=uint32(1)
  Constant1 : Constant  Value=[0:5]  OutDataTypeStr=uint32
  Constant2 : Constant  Value=[0:5]  OutDataTypeStr=uint32
  Constant3 : Constant  Value=[0:5]  OutDataTypeStr=uint32
  Constant4 : Constant  Value=uint32(1)
  Constant5 : Constant  Value=uint32(1)
  DamageCase3 : InportShadow  Port=2
  DamageCase4 : InportShadow  Port=2
  PreLookup Index Search : simulink_need_slupdate/PreLookup Index Search  bpData=Aero.dC6_damage.ddscale.alpha  searchMode=Binary Search  cacheBpFlag=on  outputFlag=off  IndexDataType=uint32  extrapMode=Linear Extrapolation  rangeErrorMode=None
      settings: SourceProductBaseCode=SL
  Subtract : Sum  Inputs=+-
  Subtract1 : Sum  Inputs=+-
  Subtract2 : Sum  Inputs=+-
  p : simulink_need_slupdate/Interpolation (n-D) using PreLookup  numDimsPopupSelect=3  explicitNumDims=2  table=squeeze(Aero.dC6_damage.ddscale.data(:,:,1,:))  interpMethod=Linear  extrapMethod=None - Clip  rangeErrorMode=None  NumSelectionDims=2
      settings: SourceProductBaseCode=SL
  q : simulink_need_slupdate/Interpolation (n-D) using PreLookup  numDimsPopupSelect=3  explicitNumDims=2  table=squeeze(Aero.dC6_damage.ddscale.data(:,:,2,:))  interpMethod=Linear  extrapMethod=None - Clip  rangeErrorMode=None  NumSelectionDims=2
      settings: SourceProductBaseCode=SL
  r : simulink_need_slupdate/Interpolation (n-D) using PreLookup  numDimsPopupSelect=3  explicitNumDims=2  table=squeeze(Aero.dC6_damage.ddscale.data(:,:,3,:))  interpMethod=Linear  extrapMethod=None - Clip  rangeErrorMode=None  NumSelectionDims=2
      settings: SourceProductBaseCode=SL
  Scaling_r : Outport
  Scaling_q : Outport  Port=2
  Scaling_p : Outport  Port=3
  wires:
  DamageCase4/1 -> Subtract2/1
  Subtract2/1 -> p/2
  DamageCase3/1 -> Subtract1/1
  Subtract1/1 -> q/2
  Constant5/1 -> Subtract2/2
  Constant4/1 -> Subtract1/2
  DamageCase/1 -> Subtract/1
  Subtract/1 -> r/2
  Constant/1 -> Subtract/2
  alpha/1 -> PreLookup Index Search/1
  r/1 -> Scaling_r/1
  PreLookup Index Search/1 -> r/1, q/1, p/1
  q/1 -> Scaling_q/1
  p/1 -> Scaling_p/1
  Constant1/1 -> r/3
  Constant2/1 -> q/3
  Constant3/1 -> p/3

== system gtm_design/GTM_T2/Aero/Dynamic Derviatives/Forced Oscillation with Damage Increments/Forced Oscillation ==
  alpha : Inport
  pqr : Inport  Port=2
  Assignment to Lateral : Assignment  IndexMode=Zero-based  IndexOptions=Index vector (dialog)  Indices=[1 3 5]  OutputSizes=[1 1]
  Assignment to Lateral1 : Assignment  IndexMode=Zero-based  IndexOptions=Index vector (dialog)  Indices=[1 3 5]  OutputSizes=[1 1]
  Assignment to Longitudinal : Assignment  IndexMode=Zero-based  IndexOptions=Index vector (dialog)  Indices=[0 2 4]  OutputSizes=[1 1]
  Constant : Constant  Value=zeros(6,1)
  Constant1 : Constant  Value=[0:2]  OutDataTypeStr=uint32
  Constant2 : Constant  Value=[0:2]  OutDataTypeStr=uint32
  Constant3 : Constant  Value=[0:2]  OutDataTypeStr=uint32
  Constant4 : Constant  Value=zeros(6,1)
  Constant5 : Constant  Value=zeros(6,1)
  Demux : Demux  Outputs=3
  PreLookup Index Search : simulink_need_slupdate/PreLookup Index Search  bpData=Aero.dC3_q.alpha  searchMode=Binary Search  cacheBpFlag=on  outputFlag=off  IndexDataType=uint32  extrapMode=Linear Extrapolation  rangeErrorMode=None
      settings: SourceProductBaseCode=SL
  PreLookup Index Search1 : simulink_need_slupdate/PreLookup Index Search  bpData=Aero.dC3_r.rhat  searchMode=Binary Search  cacheBpFlag=on  outputFlag=off  IndexDataType=uint32  extrapMode=Linear Extrapolation  rangeErrorMode=None
      settings: SourceProductBaseCode=SL
  PreLookup Index Search2 : simulink_need_slupdate/PreLookup Index Search  bpData=Aero.dC3_p.phat  searchMode=Binary Search  cacheBpFlag=on  outputFlag=off  IndexDataType=uint32  extrapMode=Linear Extrapolation  rangeErrorMode=None
      settings: SourceProductBaseCode=SL
  PreLookup Index Search3 : simulink_need_slupdate/PreLookup Index Search  bpData=Aero.dC3_q.qhat  searchMode=Binary Search  cacheBpFlag=on  outputFlag=off  IndexDataType=uint32  extrapMode=Linear Extrapolation  rangeErrorMode=None
      settings: SourceProductBaseCode=SL
  PreLookup Index Search4 : simulink_need_slupdate/PreLookup Index Search  bpData=Aero.dC3_p.alpha  searchMode=Binary Search  cacheBpFlag=on  outputFlag=off  IndexDataType=uint32  extrapMode=Linear Extrapolation  rangeErrorMode=None
      settings: SourceProductBaseCode=SL
  PreLookup Index Search5 : simulink_need_slupdate/PreLookup Index Search  bpData=Aero.dC3_r.alpha  searchMode=Binary Search  cacheBpFlag=on  outputFlag=off  IndexDataType=uint32  extrapMode=Linear Extrapolation  rangeErrorMode=None
      settings: SourceProductBaseCode=SL
  pitch : simulink_need_slupdate/Interpolation (n-D) using PreLookup  numDimsPopupSelect=3  explicitNumDims=2  table=Aero.dC3_q.data  interpMethod=Linear  extrapMethod=None - Clip  rangeErrorMode=None  NumSelectionDims=1
      settings: SourceProductBaseCode=SL
  roll : simulink_need_slupdate/Interpolation (n-D) using PreLookup  numDimsPopupSelect=3  explicitNumDims=2  table=Aero.dC3_p.data  interpMethod=Linear  extrapMethod=None - Clip  rangeErrorMode=None  NumSelectionDims=1
      settings: SourceProductBaseCode=SL
  yaw : simulink_need_slupdate/Interpolation (n-D) using PreLookup  numDimsPopupSelect=3  explicitNumDims=2  table=Aero.dC3_r.data  interpMethod=Linear  extrapMethod=None - Clip  rangeErrorMode=None  NumSelectionDims=1
      settings: SourceProductBaseCode=SL
  dC6_p : Outport
  dC6_q : Outport  Port=2
  dC6_r : Outport  Port=3
  wires:
  alpha/1 -> PreLookup Index Search4/1, PreLookup Index Search5/1, PreLookup Index Search/1
  pqr/1 -> Demux/1
  Constant1/1 -> pitch/3
  Demux/2 -> PreLookup Index Search3/1
  Demux/1 -> PreLookup Index Search2/1
  Demux/3 -> PreLookup Index Search1/1
  Constant2/1 -> roll/3
  Constant3/1 -> yaw/3
  Constant/1 -> Assignment to Longitudinal/1
  pitch/1 -> Assignment to Longitudinal/2
  roll/1 -> Assignment to Lateral/2
  Constant4/1 -> Assignment to Lateral/1
  Constant5/1 -> Assignment to Lateral1/1
  yaw/1 -> Assignment to Lateral1/2
  PreLookup Index Search1/1 -> yaw/2
  PreLookup Index Search2/1 -> roll/2
  PreLookup Index Search3/1 -> pitch/2
  Assignment to Lateral/1 -> dC6_p/1
  Assignment to Lateral1/1 -> dC6_r/1
  Assignment to Longitudinal/1 -> dC6_q/1
  PreLookup Index Search/1 -> pitch/1
  PreLookup Index Search4/1 -> roll/1
  PreLookup Index Search5/1 -> yaw/1

== system gtm_design/GTM_T2/Aero/Dynamic Derviatives/Forced Oscillation with Damage Increments/Normalize ==
  pqr : Inport
  TAS : Inport  Port=2
  AC_Params : Inport  Port=3
  Bus Selector2 : BusSelector  OutputSignals=B,Cbar,B
  Gain : Gain  Gain=2*(1.689)
  Mux : Mux  Inputs=3
  Product3 : Product  Inputs=**/  RndMeth=Zero
  Saturation1 : Saturate  UpperLimit=10000  LowerLimit=1
  pqrhat : Outport
  wires:
  Mux/1 -> Product3/2
  Bus Selector2/3 -> Mux/3  "<B>"
  Bus Selector2/2 -> Mux/2  "<Cbar>"
  Bus Selector2/1 -> Mux/1  "<B>"
  Product3/1 -> pqrhat/1
  Gain/1 -> Product3/3
  pqr/1 -> Product3/1
  Saturation1/1 -> Gain/1
  AC_Params/1 -> Bus Selector2/1
  TAS/1 -> Saturation1/1

== system gtm_design/GTM_T2/Aero/Dynamic Derviatives/Rotary Blended UnDamaged Case/Forced Oscillation ==
  alpha : Inport
  pqr : Inport  Port=2
  Assignment to Lateral : Assignment  IndexMode=Zero-based  IndexOptions=Index vector (dialog)  Indices=[1 3 5]  OutputSizes=[1 1]
  Assignment to Lateral1 : Assignment  IndexMode=Zero-based  IndexOptions=Index vector (dialog)  Indices=[1 3 5]  OutputSizes=[1 1]
  Assignment to Longitudinal : Assignment  IndexMode=Zero-based  IndexOptions=Index vector (dialog)  Indices=[0 2 4]  OutputSizes=[1 1]
  Constant : Constant  Value=zeros(6,1)
  Constant1 : Constant  Value=[0:2]  OutDataTypeStr=uint32
  Constant2 : Constant  Value=[0:2]  OutDataTypeStr=uint32
  Constant3 : Constant  Value=[0:2]  OutDataTypeStr=uint32
  Constant4 : Constant  Value=zeros(6,1)
  Constant5 : Constant  Value=zeros(6,1)
  Demux : Demux  Outputs=3
  PreLookup Index Search : simulink_need_slupdate/PreLookup Index Search  bpData=Aero.dC3_q.alpha  searchMode=Binary Search  cacheBpFlag=on  outputFlag=off  IndexDataType=uint32  extrapMode=Linear Extrapolation  rangeErrorMode=None
      settings: SourceProductBaseCode=SL
  PreLookup Index Search1 : simulink_need_slupdate/PreLookup Index Search  bpData=Aero.dC3_r.rhat  searchMode=Binary Search  cacheBpFlag=on  outputFlag=off  IndexDataType=uint32  extrapMode=Linear Extrapolation  rangeErrorMode=None
      settings: SourceProductBaseCode=SL
  PreLookup Index Search2 : simulink_need_slupdate/PreLookup Index Search  bpData=Aero.dC3_p.phat  searchMode=Binary Search  cacheBpFlag=on  outputFlag=off  IndexDataType=uint32  extrapMode=Linear Extrapolation  rangeErrorMode=None
      settings: SourceProductBaseCode=SL
  PreLookup Index Search3 : simulink_need_slupdate/PreLookup Index Search  bpData=Aero.dC3_q.qhat  searchMode=Binary Search  cacheBpFlag=on  outputFlag=off  IndexDataType=uint32  extrapMode=Linear Extrapolation  rangeErrorMode=None
      settings: SourceProductBaseCode=SL
  PreLookup Index Search4 : simulink_need_slupdate/PreLookup Index Search  bpData=Aero.dC3_p.alpha  searchMode=Binary Search  cacheBpFlag=on  outputFlag=off  IndexDataType=uint32  extrapMode=Linear Extrapolation  rangeErrorMode=None
      settings: SourceProductBaseCode=SL
  PreLookup Index Search5 : simulink_need_slupdate/PreLookup Index Search  bpData=Aero.dC3_r.alpha  searchMode=Binary Search  cacheBpFlag=on  outputFlag=off  IndexDataType=uint32  extrapMode=Linear Extrapolation  rangeErrorMode=None
      settings: SourceProductBaseCode=SL
  pitch : simulink_need_slupdate/Interpolation (n-D) using PreLookup  numDimsPopupSelect=3  explicitNumDims=2  table=Aero.dC3_q.data  interpMethod=Linear  extrapMethod=Linear  rangeErrorMode=None  NumSelectionDims=1
      settings: SourceProductBaseCode=SL
  roll : simulink_need_slupdate/Interpolation (n-D) using PreLookup  numDimsPopupSelect=3  explicitNumDims=2  table=Aero.dC3_p.data  interpMethod=Linear  extrapMethod=Linear  rangeErrorMode=None  NumSelectionDims=1
      settings: SourceProductBaseCode=SL
  yaw : simulink_need_slupdate/Interpolation (n-D) using PreLookup  numDimsPopupSelect=3  explicitNumDims=2  table=Aero.dC3_r.data  interpMethod=Linear  extrapMethod=Linear  rangeErrorMode=None  NumSelectionDims=1
      settings: SourceProductBaseCode=SL
  dC6_p : Outport
  dC6_q : Outport  Port=2
  dC6_r : Outport  Port=3
  wires:
  alpha/1 -> PreLookup Index Search4/1, PreLookup Index Search5/1, PreLookup Index Search/1
  pqr/1 -> Demux/1
  Constant1/1 -> pitch/3
  Demux/2 -> PreLookup Index Search3/1
  Demux/1 -> PreLookup Index Search2/1
  Demux/3 -> PreLookup Index Search1/1
  Constant2/1 -> roll/3
  Constant3/1 -> yaw/3
  Constant/1 -> Assignment to Longitudinal/1
  pitch/1 -> Assignment to Longitudinal/2
  roll/1 -> Assignment to Lateral/2
  Constant4/1 -> Assignment to Lateral/1
  Constant5/1 -> Assignment to Lateral1/1
  yaw/1 -> Assignment to Lateral1/2
  PreLookup Index Search1/1 -> yaw/2
  PreLookup Index Search2/1 -> roll/2
  PreLookup Index Search3/1 -> pitch/2
  Assignment to Lateral/1 -> dC6_p/1
  Assignment to Lateral1/1 -> dC6_r/1
  Assignment to Longitudinal/1 -> dC6_q/1
  PreLookup Index Search/1 -> pitch/1
  PreLookup Index Search4/1 -> roll/1
  PreLookup Index Search5/1 -> yaw/1

== system gtm_design/GTM_T2/Aero/Dynamic Derviatives/Rotary Blended UnDamaged Case/Rotary Balance ==
  alpha : Inport
  beta : Inport  Port=2
  w : Inport  Port=3
  Constant1 : Constant  Value=[0:5]  OutDataTypeStr=uint32
  PreLookup Index Search : simulink_need_slupdate/PreLookup Index Search  bpData=Aero.dC6_w.alpha  searchMode=Binary Search  cacheBpFlag=on  outputFlag=off  IndexDataType=uint32  extrapMode=Linear Extrapolation  rangeErrorMode=None
      settings: SourceProductBaseCode=SL
  PreLookup Index Search1 : simulink_need_slupdate/PreLookup Index Search  bpData=Aero.dC6_w.beta  searchMode=Binary Search  cacheBpFlag=on  outputFlag=off  IndexDataType=uint32  extrapMode=Linear Extrapolation  rangeErrorMode=None
      settings: SourceProductBaseCode=SL
  PreLookup Index Search2 : simulink_need_slupdate/PreLookup Index Search  bpData=Aero.dC6_w.what  searchMode=Binary Search  cacheBpFlag=on  outputFlag=off  IndexDataType=uint32  extrapMode=Linear Extrapolation  rangeErrorMode=None
      settings: SourceProductBaseCode=SL
  TableLookup : simulink_need_slupdate/Interpolation (n-D) using PreLookup  numDimsPopupSelect=4  explicitNumDims=2  table=Aero.dC6_w.data  interpMethod=Linear  extrapMethod=Linear  rangeErrorMode=None  NumSelectionDims=1
      settings: SourceProductBaseCode=SL
  dC6 : Outport
  wires:
  PreLookup Index Search/1 -> TableLookup/1
  beta/1 -> PreLookup Index Search1/1
  alpha/1 -> PreLookup Index Search/1
  TableLookup/1 -> dC6/1
  Constant1/1 -> TableLookup/4
  w/1 -> PreLookup Index Search2/1
  PreLookup Index Search1/1 -> TableLookup/3
  PreLookup Index Search2/1 -> TableLookup/2

== system gtm_design/GTM_T2/Sensors/Air Data/First Order Filter/Enabled Subsystem ==
  In : Inport
  tau : Inport  Port=2
  Enable : EnablePort
  Divide : Product  Inputs=*/
  Integrator : Integrator  InitialConditionSource=external  UpperSaturationLimit=POS_hi  LowerSaturationLimit=POS_lo
  Sum : Sum  Inputs=-+|  InputSameDT=on  SaturateOnIntegerOverflow=on  OutDataTypeStr=Inherit: Same as first input
  Out : Outport
  wires:
  Sum/1 -> Divide/1  "Error"
  In/1 -> Sum/2, Integrator/2
  Integrator/1 -> Out/1, Sum/1  "Y"
  tau/1 -> Divide/2
  Divide/1 -> Integrator/1  "Ydot"
